simulink model "servo_drive_physics"  (R2023b)
settings: Solver=ode1  StartTime=0.0  StopTime=Tend  FixedStep=dt  RelTol=1e-3
model workspace (MAT data in the model file):
  Ilim = 3
  Jt = 1e-06
  Kd = 0
  Ke = 0.00568713663315
  Ki = 1.5
  KiOn = 1
  KidDt = 7.03341638863e-05
  Kp = 0.3
  Kpd = 0.00703341638863
  Kt = 0.00568713663315
  N = 100
  R = 1.6
  TLbase = 0
  Tend = 5
  Tf = 0.01
  Ts = 0.1
  Vs = 11.1
  accDt = 0.523598775598
  aw = 1
  b = 2.41369575255e-06
  closedLoop = 1
  dt = 0.001
  kU = 10.471975512
  measSel = 1
  nLat = 70
  olProfile = [0 60]
  qCnt = 1
  qSpd = 4.615
  spProfile = [0 60]
  tDist = 3
  uMax = 180
  wMax = 1884.95559215
libraries: simulink x3
settings Model: Creator=odyssix  LastModifiedBy=odyssix
settings ModelReferenceCC: UpdateModelReferenceTargets=IfOutOfDate
settings RTWCC: GPUComputeCapability=5.0
settings ConfigComp: CovBoundaryAbsTol=1.0e-5

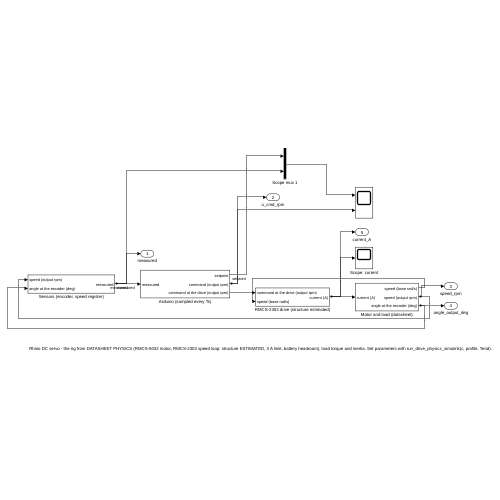
[thumbnail: Simulink's stored preview of the top-level diagram]
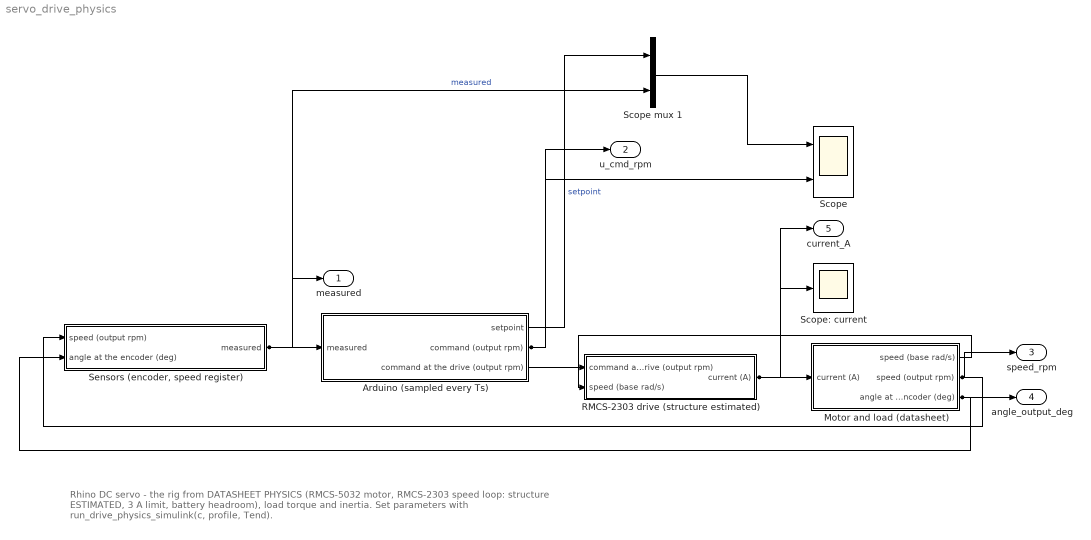
== system servo_drive_physics ==
  note: Rhino DC servo - the rig from DATASHEET PHYSICS (RMCS-5032 motor, RMCS-2303 speed loop: structure ESTIMATED, 3 A limit, battery headroom), load torque and inertia. Set parameters with run_drive_physics_simulink(c, profile, Tend).
  Arduino (sampled every Ts) : Subsystem
  Motor and load (datasheet) : Subsystem
  RMCS-2303 drive (structure estimated) : Subsystem
  Scope : Scope  NumInputPorts=2
  Scope mux 1 : Mux  Inputs=2
  Scope: current : Scope
  "Sensors (encoder, speed register)" : Subsystem
  measured : Outport
  u_cmd_rpm : Outport  Port=2
  speed_rpm : Outport  Port=3
  angle_output_deg : Outport  Port=4
  current_A : Outport  Port=5
  wires:
  Motor and load (datasheet)/3(angle at the encoder (deg)) -> angle_output_deg/1, "Sensors (encoder, speed register)"/2(angle at the encoder (deg))
  RMCS-2303 drive (structure estimated)/1(current (A)) -> Scope: current/1, Motor and load (datasheet)/1(current (A)), current_A/1
  Motor and load (datasheet)/2(speed (output rpm)) -> speed_rpm/1, "Sensors (encoder, speed register)"/1(speed (output rpm))
  Motor and load (datasheet)/1(speed (base rad/s)) -> RMCS-2303 drive (structure estimated)/2(speed (base rad/s))
  Scope mux 1/1 -> Scope/1
  Arduino (sampled every Ts)/3(command at the drive (output rpm)) -> RMCS-2303 drive (structure estimated)/1(command at the drive (output rpm))
  Arduino (sampled every Ts)/2(command (output rpm)) -> u_cmd_rpm/1, Scope/2
  Arduino (sampled every Ts)/1(setpoint) -> Scope mux 1/1  "setpoint"
  "Sensors (encoder, speed register)"/1(measured) -> Arduino (sampled every Ts)/1(measured), Scope mux 1/2, measured/1  "measured"

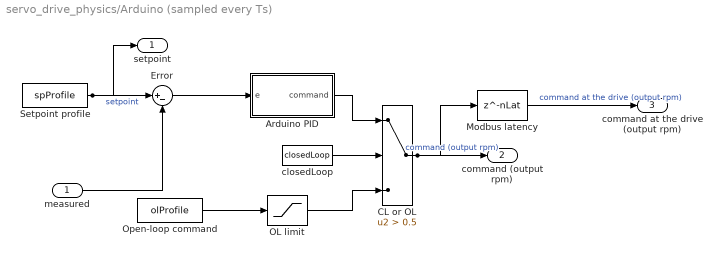
== system servo_drive_physics/Arduino (sampled every Ts) ==
  measured : Inport
  Arduino PID : Subsystem
  CL or OL : Switch  Criteria=u2 > Threshold  Threshold=0.5  SaturateOnIntegerOverflow=off  InputSameDT=off
  Error : Sum  Inputs=|+-
  Modbus latency : Delay  DelayLength=nLat  SampleTime=dt
  OL limit : Saturate  UpperLimit=uMax  LowerLimit=-uMax
  Open-loop command : FromWorkspace  VariableName=olProfile  SampleTime=Ts  Interpolate=off  OutputAfterFinalValue=Holding final value
  Setpoint profile : FromWorkspace  VariableName=spProfile  SampleTime=Ts  Interpolate=off  OutputAfterFinalValue=Holding final value
  closedLoop : Constant  Value=closedLoop
  setpoint : Outport
  command (output rpm) : Outport  Port=2
  command at the drive (output rpm) : Outport  Port=3
  wires:
  closedLoop/1 -> CL or OL/2
  Arduino PID/1(command) -> CL or OL/1
  CL or OL/1 -> Modbus latency/1, command (output rpm)/1  "command (output rpm)"
  OL limit/1 -> CL or OL/3
  Error/1 -> Arduino PID/1(e)
  Modbus latency/1 -> command at the drive (output rpm)/1  "command at the drive (output rpm)"
  Open-loop command/1 -> OL limit/1
  measured/1 -> Error/2
  Setpoint profile/1 -> setpoint/1, Error/1  "setpoint"

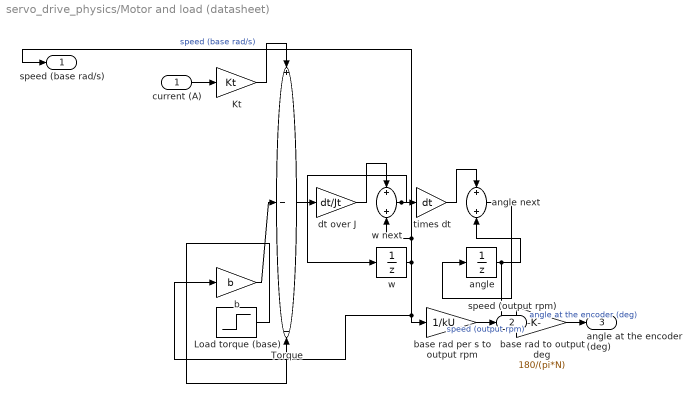
== system servo_drive_physics/Motor and load (datasheet) ==
  current (A) : Inport
  Kt : Gain  Gain=Kt
  Load torque (base) : Step  Time=tDist  After=TLbase  SampleTime=dt
  Torque : Sum  Inputs=+--
  angle : UnitDelay  SampleTime=dt
  angle next : Sum
  b : Gain  Gain=b
  base rad per s to output rpm : Gain  Gain=1/kU
  base rad to output deg : Gain  Gain=180/(pi*N)
  dt over J : Gain  Gain=dt/Jt
  times dt : Gain  Gain=dt
  w : UnitDelay  SampleTime=dt
  w next : Sum
  speed (base rad/s) : Outport
  speed (output rpm) : Outport  Port=2
  angle at the encoder (deg) : Outport  Port=3
  wires:
  angle next/1 -> angle/1
  Torque/1 -> dt over J/1
  angle/1 -> angle next/2, base rad to output deg/1
  Kt/1 -> Torque/1
  Load torque (base)/1 -> Torque/3
  times dt/1 -> angle next/1
  dt over J/1 -> w next/1
  current (A)/1 -> Kt/1
  base rad to output deg/1 -> angle at the encoder (deg)/1  "angle at the encoder (deg)"
  base rad per s to output rpm/1 -> speed (output rpm)/1  "speed (output rpm)"
  b/1 -> Torque/2
  w next/1 -> w/1, times dt/1
  w/1 -> speed (base rad/s)/1, w next/2, b/1, base rad per s to output rpm/1  "speed (base rad/s)"

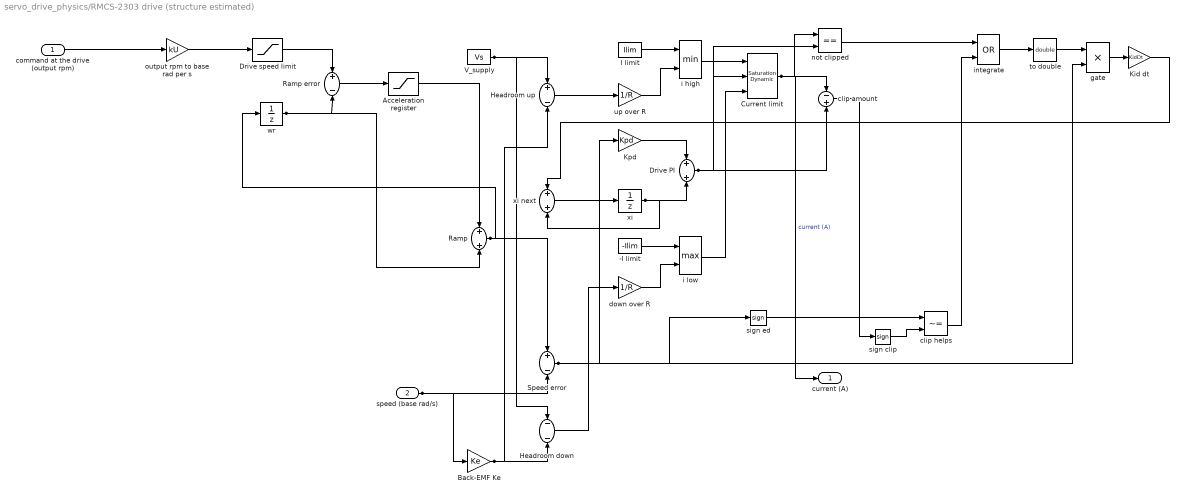
== system servo_drive_physics/RMCS-2303 drive (structure estimated) ==
  command at the drive (output rpm) : Inport
  speed (base rad/s) : Inport  Port=2
  -I limit : Constant  Value=-Ilim
  Acceleration register : Saturate  UpperLimit=accDt  LowerLimit=-accDt
  Back-EMF Ke : Gain  Gain=Ke
  Current limit : simulink/Discontinuities/Saturation Dynamic  OutMin=[]  OutMax=[]  OutDataTypeStr=Inherit: Same as second input  OutDataType=fixdt(1, 16)  OutScaling=2^-10  DoSatur=off
      settings: LibrarySourceBlock=|
      | simulink/Discontinuities/Saturation
      | Dynamic
  Drive PI : Sum
  Drive speed limit : Saturate  UpperLimit=wMax  LowerLimit=-wMax
  Headroom down : Sum  Inputs=--
  Headroom up : Sum  Inputs=+-
  I limit : Constant  Value=Ilim
  Kid dt : Gain  Gain=KidDt
  Kpd : Gain  Gain=Kpd
  Ramp : Sum
  Ramp error : Sum  Inputs=+-
  Speed error : Sum  Inputs=+-
  V_supply : Constant  Value=Vs
  clip amount : Sum  Inputs=-+
  clip helps : RelationalOperator  Operator=~=  OutDataTypeStr=boolean  RndMeth=Simplest  InputSameDT=off
  down over R : Gain  Gain=1/R
  gate : Product
  i high : MinMax  Inputs=2
  i low : MinMax  Function=max  Inputs=2
  integrate : Logic  Operator=OR  AllPortsSameDT=off  OutDataTypeStr=boolean
  not clipped : RelationalOperator  Operator===  OutDataTypeStr=boolean  RndMeth=Simplest  InputSameDT=off
  output rpm to base rad per s : Gain  Gain=kU
  sign clip : Signum
  sign ed : Signum
  to double : DataTypeConversion  OutDataTypeStr=double  SaturateOnIntegerOverflow=off  RndMeth=Floor
  up over R : Gain  Gain=1/R
  wr : UnitDelay  SampleTime=dt
  xi : UnitDelay  SampleTime=dt
  xi next : Sum
  current (A) : Outport
  wires:
  Kid dt/1 -> xi next/1
  to double/1 -> gate/1
  Ramp/1 -> Speed error/1, wr/1
  i high/1 -> Current limit/1
  Speed error/1 -> Kpd/1, sign ed/1, gate/2
  integrate/1 -> to double/1
  speed (base rad/s)/1 -> Back-EMF Ke/1, Speed error/2
  xi next/1 -> xi/1
  Kpd/1 -> Drive PI/1
  Acceleration register/1 -> Ramp/1
  wr/1 -> Ramp/2, Ramp error/2
  -I limit/1 -> i low/1
  V_supply/1 -> Headroom up/1, Headroom down/1
  output rpm to base rad per s/1 -> Drive speed limit/1
  Headroom up/1 -> up over R/1
  command at the drive (output rpm)/1 -> output rpm to base rad per s/1
  I limit/1 -> i high/1
  up over R/1 -> i high/2
  Back-EMF Ke/1 -> Headroom down/2, Headroom up/2
  i low/1 -> Current limit/3
  xi/1 -> Drive PI/2, xi next/2
  down over R/1 -> i low/2
  clip helps/1 -> integrate/2
  gate/1 -> Kid dt/1
  Drive speed limit/1 -> Ramp error/1
  Drive PI/1 -> Current limit/2, clip amount/2, not clipped/2
  Ramp error/1 -> Acceleration register/1
  Current limit/1 -> current (A)/1, not clipped/1, clip amount/1  "current (A)"
  Headroom down/1 -> down over R/1
  sign ed/1 -> clip helps/1
  not clipped/1 -> integrate/1
  clip amount/1 -> sign clip/1
  sign clip/1 -> clip helps/2

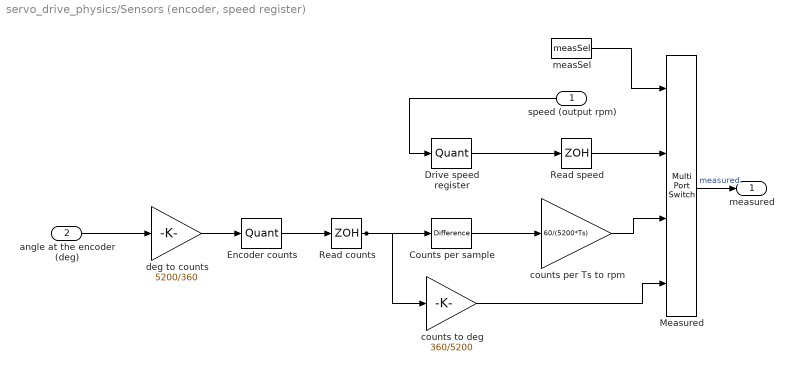
== system servo_drive_physics/Sensors (encoder, speed register) ==
  speed (output rpm) : Inport
  angle at the encoder (deg) : Inport  Port=2
  Counts per sample : simulink/Discrete/Difference  ICPrevInput=0.0  OutMin=[]  OutMax=[]  OutDataType=fixdt(1, 16)  OutScaling=2^-10  DoSatur=off
  Drive speed register : Quantizer  QuantizationInterval=qSpd
  Encoder counts : Quantizer  QuantizationInterval=qCnt
  Measured : MultiPortSwitch  SaturateOnIntegerOverflow=off  InputSameDT=off
  Read counts : ZeroOrderHold  SampleTime=Ts
  Read speed : ZeroOrderHold  SampleTime=Ts
  counts per Ts to rpm : Gain  Gain=60/(5200*Ts)
  counts to deg : Gain  Gain=360/5200
  deg to counts : Gain  Gain=5200/360
  measSel : Constant  Value=measSel
  measured : Outport
  wires:
  counts per Ts to rpm/1 -> Measured/3
  Read speed/1 -> Measured/2
  measSel/1 -> Measured/1
  speed (output rpm)/1 -> Drive speed register/1
  Counts per sample/1 -> counts per Ts to rpm/1
  counts to deg/1 -> Measured/4
  Read counts/1 -> counts to deg/1, Counts per sample/1
  Drive speed register/1 -> Read speed/1
  deg to counts/1 -> Encoder counts/1
  Measured/1 -> measured/1  "measured"
  Encoder counts/1 -> Read counts/1
  angle at the encoder (deg)/1 -> deg to counts/1

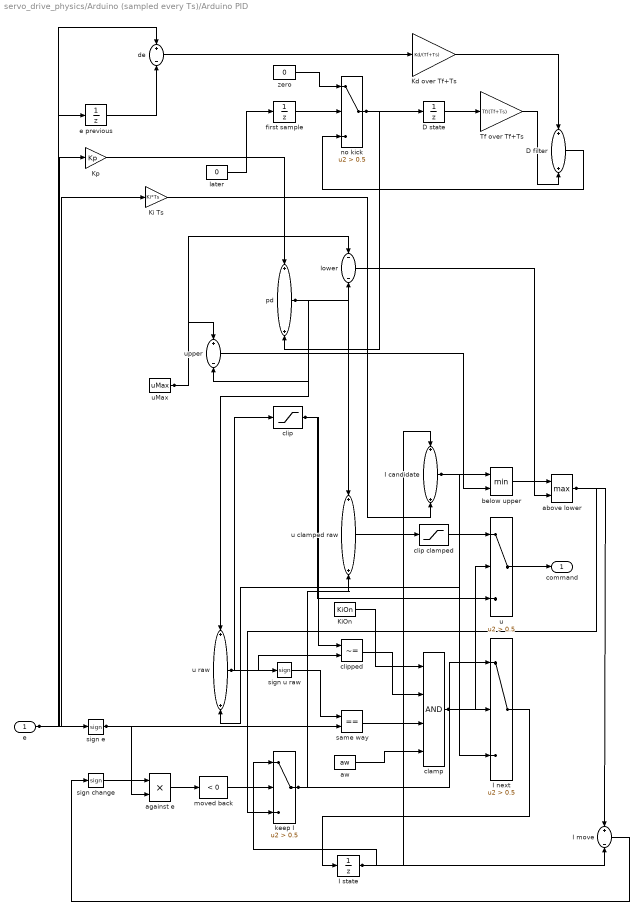
== system servo_drive_physics/Arduino (sampled every Ts)/Arduino PID ==
  e : Inport
  D filter : Sum
  D state : UnitDelay  SampleTime=Ts
  I candidate : Sum
  I move : Sum  Inputs=+-
  I next : Switch  Criteria=u2 > Threshold  Threshold=0.5  SaturateOnIntegerOverflow=off  InputSameDT=off
  I state : UnitDelay  SampleTime=Ts
  Kd over Tf+Ts : Gain  Gain=Kd/(Tf+Ts)
  Ki Ts : Gain  Gain=Ki*Ts
  KiOn : Constant  Value=KiOn
  Kp : Gain  Gain=Kp
  Tf over Tf+Ts : Gain  Gain=Tf/(Tf+Ts)
  above lower : MinMax  Function=max  Inputs=2
  against e : Product
  aw : Constant  Value=aw
  below upper : MinMax  Inputs=2
  clamp : Logic  Inputs=4  AllPortsSameDT=off  OutDataTypeStr=boolean
  clip : Saturate  UpperLimit=uMax  LowerLimit=-uMax
  clip clamped : Saturate  UpperLimit=uMax  LowerLimit=-uMax
  clipped : RelationalOperator  Operator=~=  OutDataTypeStr=boolean  RndMeth=Simplest  InputSameDT=off
  de : Sum  Inputs=+-
  e previous : UnitDelay  SampleTime=Ts
  first sample : UnitDelay  InitialCondition=1  SampleTime=Ts
  keep I : Switch  Criteria=u2 > Threshold  Threshold=0.5  SaturateOnIntegerOverflow=off  InputSameDT=off
  later : Constant  Value=0
  lower : Sum  Inputs=--
  moved back : simulink/Logic and Bit Operations/Compare To Constant  relop=<  const=0  OutDataTypeStr=boolean
  no kick : Switch  Criteria=u2 > Threshold  Threshold=0.5  SaturateOnIntegerOverflow=off  InputSameDT=off
  pd : Sum
  same way : RelationalOperator  Operator===  OutDataTypeStr=boolean  RndMeth=Simplest  InputSameDT=off
  sign change : Signum
  sign e : Signum
  sign u raw : Signum
  u : Switch  Criteria=u2 > Threshold  Threshold=0.5  SaturateOnIntegerOverflow=off  InputSameDT=off
  u clamped raw : Sum
  u raw : Sum
  uMax : Constant  Value=uMax
  upper : Sum  Inputs=+-
  zero : Constant  Value=0
  command : Outport
  wires:
  I move/1 -> sign change/1
  above lower/1 -> I move/1, keep I/3
  I next/1 -> I state/1
  below upper/1 -> above lower/1
  clamp/1 -> u/2, I next/2
  clip clamped/1 -> u/1
  upper/1 -> below upper/2
  u/1 -> command/1
  lower/1 -> above lower/2
  I state/1 -> I candidate/1, I move/2, keep I/1
  against e/1 -> moved back/1
  Ki Ts/1 -> I candidate/2
  no kick/1 -> D state/1, pd/2
  later/1 -> first sample/1
  Tf over Tf+Ts/1 -> D filter/2
  uMax/1 -> lower/1, upper/1
  sign e/1 -> against e/2, same way/2
  e previous/1 -> de/2
  sign u raw/1 -> same way/1
  u raw/1 -> sign u raw/1, clip/1, clipped/2
  Kp/1 -> pd/1
  sign change/1 -> against e/1
  clipped/1 -> clamp/2
  de/1 -> Kd over Tf+Ts/1
  e/1 -> sign e/1, Kp/1, e previous/1, Ki Ts/1, de/1
  I candidate/1 -> I next/3, u raw/2, below upper/1
  zero/1 -> no kick/1
  pd/1 -> u clamped raw/1, lower/2, upper/2, u raw/1
  first sample/1 -> no kick/2
  Kd over Tf+Ts/1 -> D filter/1
  D state/1 -> Tf over Tf+Ts/1
  clip/1 -> clipped/1, u/3
  moved back/1 -> keep I/2
  u clamped raw/1 -> clip clamped/1
  D filter/1 -> no kick/3
  keep I/1 -> I next/1, u clamped raw/2
  KiOn/1 -> clamp/1
  same way/1 -> clamp/3
  aw/1 -> clamp/4
